simulink model "WindFarmDFIG"  (R2024a)
settings: Solver=FixedStepDiscrete  StartTime=0.0  StopTime=0.2  RelTol=1e-3
PreLoadFcn:
  | Ts=5e-6;
InitFcn:
  | xInitial = WindFarmDFIGInit;
  | Ts=5e-6;
undefined symbols (not defined in the file): D1, D11, Delta, DiscIntNeverNeededParam, find_system, level
libraries: powerlib_extras x38, spsThreePhaseVIMeasurementLib x6, simulink_extras x6, spsThreePhaseTransformerTwoWindingsLib x3, spsSeriesRLCBranchLib x2, spsUniversalBridgeLib x2, spsGroundLib x2, spsThreePhaseProgrammableVoltageSourceLib x1, spsThreePhaseMutualInductanceZ1Z0Lib x1, spsThreePhasePISectionLineLib x1, spsAsynchronousMachinepuUnitsLib x1, spsThreePhaseSeriesRLCBranchLib x1
(part 1 of 3)
settings Model: FPTRunName=Active  Creator=The MathWorks, Inc.  LastModifiedBy=TUF
settings SolverCC: AlgebraicLoopSolver=TrustRegion
settings DataIOCC: LimitDataPoints=on  LoadInitialState=on  SaveFormat=StructureWithTime  SaveOutput=off  SaveTime=off  ReturnWorkspaceOutputs=off
settings OptimizationCC: ExpressionDepthLimit=2147483647  InitFltsAndDblsToZero=on  LifeSpan=inf
settings DebuggingCC: SaveWithParameterizedLinksMsg=none  UnderspecifiedInitializationDetection=Classic  MergeDetectMultiDrivingBlocksExec=none  SignalResolutionControl=TryResolveAllWithWarning  SolverPrmCheckMsg=warning  FcnCallInpInsideContextMsg=warning  UnconnectedInputMsg=warning  UnconnectedOutputMsg=warning  StateNameClashWarn=warning  SubsystemReferenceDiagnosticForUnitTest=warning  SFUnexpectedBacktrackingDiag=warning  SFNoUnconditionalDefaultTransitionDiag=warning  SFExecutionAtInitializationDiag=none  ArithmeticOperatorsInVariantConditions=warning
settings HardwareCC: ProdBitPerPointer=32  ProdBitPerSizeT=32  ProdBitPerPtrDiffT=32  ProdLargestAtomicFloat=None  ProdIntDivRoundTo=Undefined  ProdEndianess=Unspecified  ProdWordSize=32  ProdHWDeviceType=32-bit Generic
settings ModelReferenceCC: EnableRefExpFcnMdlSchedulingChecks=on  PropagateSignalLabelsOutOfModel=off
settings SFSimCC: SimUseLocalCustomCode=off  CustomCodeUndefinedFunction=UseInterfaceOnly
settings RTWCC: RTWUseLocalCustomCode=off  GPUComputeCapability=3.5  DLArmComputeVersion=19.05
settings CodeAppCC: StateflowObjectComments=on
settings GRTTargetCC: TargetFcnLib=ansi_tfl_tmw.mat  TargetLangStandard=C89/C90 (ANSI)  CombineOutputUpdateFcns=off  GRTInterface=on
settings ConfigComp: CovMetricSettings=dw  CovSaveCumulativeToWorkspaceVar=on  CovSaveSingleToWorkspaceVar=on  CovExternalEMLEnable=off  CovSFcnEnable=off  CovBoundaryAbsTol=1.0e-5
settings SimscapeCC: SimscapeNormalizeSystem=off

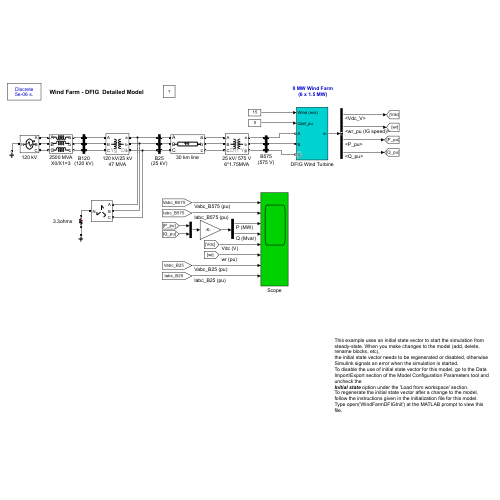
[thumbnail: Simulink's stored preview of the top-level diagram]
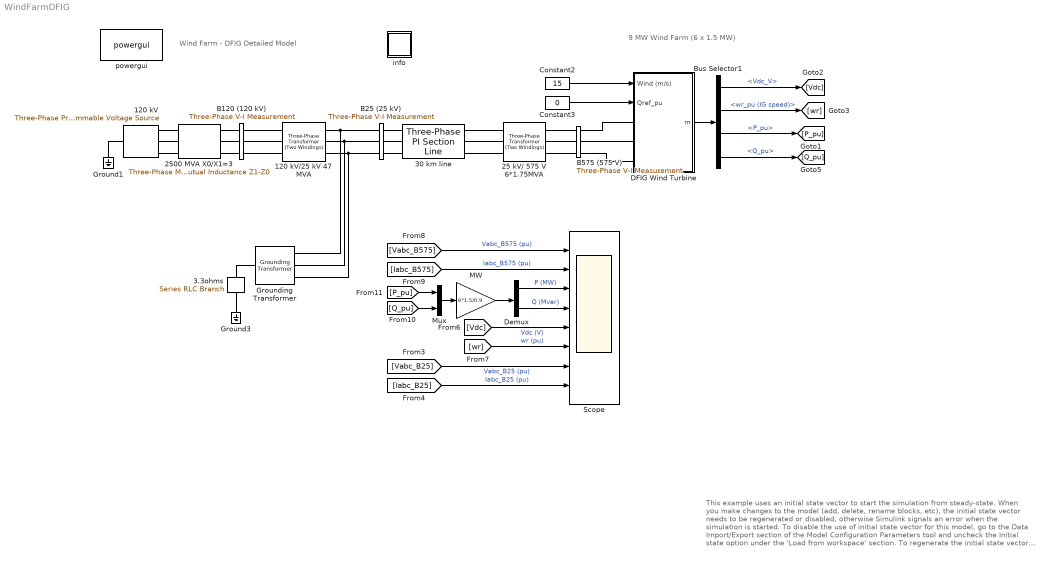
== system WindFarmDFIG ==
  note: 9 MW Wind Farm
      | (6 x 1.5 MW)
  note: Wind Farm - DFIG Detailed Model
  note: This example uses an initial state vector to start the simulation from steady-state. When you make changes to the model (add, delete, rename blocks, etc),
      | the initial state vector needs to be regenerated or disabled, otherwise Simulink signals an error when the simulation is started.
      | To disable the use of initial state vector for this model, go to the Data Import/Export section of the Model Configuration Parameters tool and uncheck the
      | Initial state option under the 'Load from workspace' section.
      | To regenerate the initial state vector after a change to the model, follow the instructions given in the initialization file for this model.
      | Type open('WindFarmDFIGInit') at the MATLAB prompt to view this file.
  120 kV : spsThreePhaseProgrammableVoltageSourceLib/Three-Phase Programmable Voltage Source  PositiveSequence=[120e3 0 60]  VariationEntity=Amplitude  VariationType=Table of time-amplitude pairs  VariationTypeAlt=Step  VariationStep=-0.2  VariationRate=10  VariationMagnitude=0.3  VariationFrequency=2  VariationTiming=[0.05 0.05+5/60]  VariationPhaseA=off  Amplitudes=[1 0.5 1.0]  TimeValues=[0 0.03 0.13]  HarmonicGeneration=off  HarmonicA=[1 -0.1 0 2]  HarmonicB=[2 0.15 35 2]*0  Timing="[0.1  2]"  BusType=swing  Pref=0  Qref=0  Qmin=-inf  Qmax=inf
  120 kV/25 kV 47 MVA : spsThreePhaseTransformerTwoWindingsLib/Three-Phase Transformer (Two Windings)  Winding1Connection=Yg  Winding2Connection=Delta (D1)  CoreType=Three single-phase transformers  SetSaturation=off  Hysteresis=off  DataFile='basic_model'  SetInitialFlux=off  Measurements=None  UNITS=pu  NominalPower=[47e6 60 ]  Winding1="[ 120e3  0.08/30   0.08 ]"  Winding2="[ 25e3  0.08/30  0.08]"  Rm=500  Lm=500  L0=0.5  Saturation="[ 0,0  ;  0.005,1.2  ;  1.0,1.4 ]"  InitialFluxes=[ 0.8 , -0.8 , 0.7 ]  BreakLoop=off  DiscreteSolver=Trapezoidal iterative  DataType=off  TransfoNumber=0
  25 kV/ 575 V 6*1.75MVA : spsThreePhaseTransformerTwoWindingsLib/Three-Phase Transformer (Two Windings)  Winding1Connection=Delta (D11)  Winding2Connection=Yg  CoreType=Three single-phase transformers  SetSaturation=off  Hysteresis=off  DataFile='hysteresis'  SetInitialFlux=off  Measurements=None  UNITS=pu  NominalPower="[1.75e6*6  60]"  Winding1=[25e3 , 0.025/30 , 0.025]  Winding2=[ 575, 0.025/30 , 0.025]  Rm=500  Lm=inf  L0=0.5  Saturation=[ 0,0 ; 0.0024,1.2 ; 1.0,1.52 ]  InitialFluxes=[ 0.8 , -0.8 , 0.7 ]  BreakLoop=off  DiscreteSolver=Trapezoidal iterative  DataType=off  TransfoNumber=0
  2500 MVA X0/X1=3 : spsThreePhaseMutualInductanceZ1Z0Lib/Three-Phase Mutual Inductance Z1-Z0  LConnTagsString=a|b|c  RConnTagsString=A|B|C  PositiveSequence="[0.1  1.0/(2*pi*60)] *120e3^2/2500e6"  ZeroSequence="[0.3  3.0/(2*pi*60)] *120e3^2/2500e6"
      settings: AttributesFormatString=\n
  "3.3ohms " : spsSeriesRLCBranchLib/Series RLC Branch  LConnTagsString=__new0  RConnTagsString=__new0  BranchType=R  Resistance=3.3  Inductance=[]  SetiL0=off  InitialCurrent=0  Capacitance=[]  Setx0=off  InitialVoltage=0  Measurements=None
  30 km line : spsThreePhasePISectionLineLib/Three-Phase PI Section Line  LConnTagsString=a|b|c  RConnTagsString=A|B|C  Length=30  Frequency=60  Resistances=[0.1153 0.413]  Inductances=[1.05e-3 3.32e-3]  Capacitances=[11.33e-009 5.01e-009]
  B120 (120 kV) : spsThreePhaseVIMeasurementLib/Three-Phase V-I Measurement  VoltageMeasurement=no  SetLabelV=off  LabelV=Vabc_B120  Vpu=off  VpuLL=off  CurrentMeasurement=no  SetLabelI=on  LabelI=Iabc_B120  Ipu=off  Pbase=100e6  Vbase=120e3  OutputType=Complex  PhasorSimulation=off  PSBequivalent=0
  B25 (25 kV) : spsThreePhaseVIMeasurementLib/Three-Phase V-I Measurement  VoltageMeasurement=phase-to-ground  SetLabelV=on  LabelV=Vabc_B25  Vpu=on  VpuLL=off  CurrentMeasurement=yes  SetLabelI=on  LabelI=Iabc_B25  Ipu=on  Pbase=10e6  Vbase=25e3  OutputType=Complex  PhasorSimulation=off  PSBequivalent=0
  B575 (575 V) : spsThreePhaseVIMeasurementLib/Three-Phase V-I Measurement  VoltageMeasurement=phase-to-ground  SetLabelV=on  LabelV=Vabc_B575  Vpu=on  VpuLL=off  CurrentMeasurement=yes  SetLabelI=on  LabelI=Iabc_B575  Ipu=on  Pbase=6*1.5e6/0.9  Vbase=575  OutputType=Complex  PhasorSimulation=off  PSBequivalent=0
  Bus Selector1 : BusSelector  OutputSignals=Vdc_V,wr_pu (IG speed),PQ_pu.P_pu,PQ_pu.Q_pu
  Constant2 : Constant  Value=15
  Constant3 : Constant  Value=0
  DFIG Wind Turbine : Subsystem  LoadFcn=%find_system(gcs,'FollowLinks', 'on', 'LookUnderMasks', 'all');  mask(DFIG Wind Turbine){Nb_wt=6, ShowParameters=Generator data for 1 wind turbine, nom=[1.5e6/.9 575 1975 60], sta=[ 0.023 0.18], rot=[ 0.016 0.16], Lm=2.9, mec=[0.685 0.01 3], init=[ -0.2,0   0,0,0   0,0,0 ], Imax_grid_conv=0.8, RL_grid=[ 0.3 0.003], Vdc_nom=1150, C_DClink1=10000e-6, C_var_filter1=120e3, Pmec1=1.5e6, wind_speed_CpMax=11, wind0=11, DisplayTurbChar=off, H_WT=4.32, Ksh=1.11, D_mutual=1.5, w_wt0=1.2, torque0=0.83, Kdc=[8   400], Kgrid_side_cur_reg=[0.83 5], Kspeed=[3 0.6], Krotor_side_cur_reg=[0.6 8], Ki_QV=[0.05 20], Kp_pitch=[150], Kcompensation=[3 30], PWM_freq_grid=2700, PWM_freq_rotor=1620, pitch_max=27, pitch_rate=10}
      mask prompts: Nb_wt "Number of wind turbines:"; ShowParameters "Display:"; nom "Nom. power, L-L volt. and freq. [Pn (VA), Vs_nom (Vrms), Vr_nom (Vrms), fn (Hz)]:"; sta "Stator [ Rs,Lls ] (p.u.):"; rot "Rotor [ Rr',Llr' ] (p.u.):"; Lm "Magnetizing inductance Lm (p.u.):"; mec "Inertia constant, friction factor, and pairs of poles [ H(s)  F(p.u.)  p ]:"; init "Initial conditions [s  th  ias  ibs  ics  phaseas phasebs phasecs]:"; Imax_grid_conv "Grid-side converter maximum current (pu of generator nominal current):"; RL_grid "Grid-side coupling inductor [ L, R] (p.u.):"; Vdc_nom "Nominal DC bus voltage (V):"; C_DClink1 "DC bus capacitor (F):"; C_var_filter1 "Line filter capacitor (Q=50) (var):"; Pmec1 "Nominal mechanical output power (W):"; wind_speed_CpMax "Wind speed at nominal speed and at Cp max (must be between 6 m/s and 30 m/s) (m/s):"; wind0 "Initial wind speed (m/s):"; DisplayTurbChar "Display wind turbine power characteristics:"; H_WT "Wind turbine inertia constant H (s):"; Ksh "Shaft spring constant refer to high-speed shaft (pu of nominal mechanical torque/rad):"; D_mutual "Shaft mutual damping (pu of nominal mechanical torque/pu dw):"; w_wt0 "Turbine initial speed (pu of nominal speed):"; torque0 "Initial output torque (pu of nominal mechanical torque):"; Kdc "DC bus voltage regulator gains [Kp Ki]:"; Kgrid_side_cur_reg "Grid-side converter current regulator gains [Kp Ki]:"; Kspeed "Speed regulator gains [Kp Ki]:"; Krotor_side_cur_reg "Rotor-side converter current regulator gains [Kp Ki]:"; Ki_QV "Q and V regulator gains [Ki_var Ki_volt]:"; Kp_pitch "Pitch controller gain [Kp]:"; Kcompensation "Pitch compensation gains [Kp Ki]:"; PWM_freq_grid "Frequency of the grid-side PWM carrier (Hz):"; PWM_freq_rotor "Frequency of the rotor-side PWM carrier (Hz):"; pitch_max "Maximum pitch angle (deg):"; pitch_rate "Maximum rate of change of pitch angle (deg/s):"
      mask help: This block implements a model of a variable speed pitch controlled wind turbine using a doubly-fed induction generator (DFIG).
      mask init:
      | %Generator data
      | Pnom=nom(1)*Nb_wt;
      | Vnom=nom(2);
      | Vnom_r=nom(3);
      | Fnom=nom(4);
      | Rs=sta(1);
      | Lls=sta(2);
      | Rr=rot(1);
      | Llr=rot(2);
      | H=mec(1);
      | F=mec(2);
      | p=mec(3);
      | 
      | % Converters data
      | L_RL=RL_grid(1);
      | R_RL=RL_grid(2);
      | Q_filter=50;
      | C_DClink=C_DClink1*Nb_wt;
      | C_var_filter=C_var_filter1*Nb_wt;
      | 
      | % Controller data
      | Freq_filter=1000*10;   %Hz
      | Zeta_filter=0.707;
      | Mod_index_max_grid=1.1;   %Maximum value of modulation index for grid-side converter
      | Mod_index_max_rotor=2;   %Maximum value of modulation index for rotor-side converter
      | Lim_grid_side_cur_reg=1.1; %Limit for grid-side PI current regulator (pu)
      | Lim_rotor_side_cur_reg=0.1; %Limit for rotor-side PI current regulator (pu)
      | Min_var_reg=0.9; %Minimum output value for integral var regulator (pu)
      | Max_var_reg=1.1; %Maximum output value for integral var regulator (pu)
      | Max_speed_reg=1; %Maximum output value for PI speed regulator (pu)
      | Kp_dc=Kdc(1);
      | Ki_dc=Kdc(2);
      | Kp_grid_side_cur_reg=Kgrid_side_cur_reg(1);
      | Ki_grid_side_cur_reg=Kgrid_side_cur_reg(2);
      | Kp_speed=Kspeed(1);
      | Ki_speed=Kspeed(2);
      | Kp_compensation=Kcompensation(1);
      | Ki_compensation=Kcompensation(2);
      | Kp_rotor_side_cur_reg=Krotor_side_cur_reg(1);
      | Ki_rotor_side_cur_reg=Krotor_side_cur_reg(2);
      | Ki_var=Ki_QV(1);
      | Ki_volt=Ki_QV(2);
      | Iq_ref_limit_time_constant=0.3; %(s)
      | T_speed=5;      %s
      | Min_mag_flux=0.5;   %(pu)
      | Max_Idr_ref=0.9;    %(pu)
      | Speed_max=1.2;  %(pu)
      | Speed_min=0.7;  %(pu)
      | Pitch_time_constant=0.01;    %(s)
      | 
      | 
      | % Turbine data
      | Pmec=Pmec1*Nb_wt;
      | c1 = 0.6450;
      | c2 = 116;
      | c3 = .4;
      | c4 = 5;
      | c5 = 21;
      | c6 = .00912;  % Set Pmin in stall condition (does not vary with wind_speed_Pmax)
      | c7 = .08;
      | c8 = .035;
      | theta=0;
      | CpMax=.5;
      | lambda_CpMax=9.9495;
      | 
      | c1_c8=[c1 c2 c3 c4 c5 c6 c7 c8];
      |   
      | 
      | %   Cp = c1*(c6*lambda + (-c4 - c3*(2.5 + theta) + c2*(1/(lambda + ...
      | %   c7*(2.5 + theta)) - c8/(1 + (2.5 + theta)^3)))/exp(c5*(1/(lambda + ...
      | %   c7*(2.5 + theta)) - c8/(1 + (2.5 + theta)^3))))
      | 
      | 
      |         %%%%%%%%%%%%%%%%%%%%%%%%%%%%%%%%%%%%%%%%%%%%%%%%%%%%%%%%%%%%%%%%%%%%%%%%%%%
      |         % Operation at Cp max
      |         %%%%%%%%%%%%%%%%%%%%%%%%%%%%%%%%%%%%%%%%%%%%%%%%%%%%%%%%%%%%%%%%%%%%%%%%%%%
      |         
      |         rated_omegar=1.2;
      |         omegar = rated_omegar;
      |         
      |         % Enforce boundaries on wind speed
      |         % A warning could be displayed
      |         if wind_speed_CpMax < 6
      |             wind_speed_CpMax=6;
      |             disp('Warning: Wind speed at nominal speed and at Cp max has been set to 6 m/s')
      |         end
      |         if wind_speed_CpMax > 30
      |             wind_speed_CpMax=30;
      |             disp('Warning: Wind speed at nominal speed and at Cp max has been set to 30 m/s')
      |         end
      | 
      |         K1=lambda_CpMax/omegar*wind_speed_CpMax;
      |         
      |         % Calculation of K2 needed to get P equal to the requested value at
      |         % Cp max for the requested wind speed
      |         
      |         Prated=Pmec1*Nb_wt;
      |         P_rated_omegar_theta_zero=0.75;
      |         
      |         K2 = P_rated_omegar_theta_zero*Prated/(wind_speed_CpMax^3*CpMax);
      |         
      |         K1_K2=[K1 K2];
      |         
      |         %%%%%%%%%%%%%%%%%%%%%%%%%%%%%%%%%%%%%%%%%%%%%%%%%%%%%%%%%%%%%%%%%%%%%%%%%%%
      |         % End of calculation for operation at Cp max
      |         %%%%%%%%%%%%%%%%%%%%%%%%%%%%%%%%%%%%%%%%%%%%%%%%%%%%%%%%%%%%%%%%%%%%%%%%%%%
      |         
      | 
      | %%%%%%%%%%%%%%%%%%%%%%%%%%%%%%%%%%%%%%%%%%%%%%%%%%%%%%%%%%%%%%%%%%%%%%%%%%%
      | % Plot turbine characteristics
      | %%%%%%%%%%%%%%%%%%%%%%%%%%%%%%%%%%%%%%%%%%%%%%%%%%%%%%%%%%%%%%%%%%%%%%%%%%% 
      | 
      | DisplayTurbChar=get_param(gcb,'DisplayTurbChar');
      | if strcmp(DisplayTurbChar,'on')
      |     vect_theta = 0:2:30;
      |     
      |     vect_lambda = 1:0.2:30;
      |     
      |     clear Cp;
      |     
      |     for i=1:length(vect_theta)
      |      for j=1:length(vect_lambda)
      |                 Cp(i,j) = c1*(c6*vect_lambda(j) + (-c4 - c3*(2.5 + vect_theta(i)) + c2*(1/(vect_lambda(j) + ...
      |                 c7*(2.5 + vect_theta(i))) - c8/(1 + (2.5 + vect_theta(i))^3)))/exp(c5*(1/(vect_lambda(j) + ...
      |                 c7*(2.5 + vect_theta(i))) - c8/(1 + (2.5 + vect_theta(i))^3))));
      |      end
      |     end
      | 
      |     figure(1);
      |     clf;
      |     hold on;
      | 
      |     plot(vect_lambda, Cp);
      |     axis([0, 25, 0, .6]);
      |     title('Wind Turbine Cp Characteristic (pitch angle increases by step of 2 deg.)');
      |     ylabel('Cp');
      |     set(gca,'ytick',[0 .1 .2 .3 .4 .5 .6]);
      |     xlabel('Lambda');
      |     grid on;
      |     text(10.1,0.51,'Pitch angle 0 degree');
      | 
      |     hold off
      |     
      |     % Plot of the wind turbine mechanical power output (pu) lambda and Cp
      |     % characteristics against wind speed (m/s) for a range of theta.
      |     
      |     wind_speed_range = [1,.2,30];
      |     vect_wind_speed = 1:0.2:30;
      |     
      |     clear lambda;
      |     clear Cp;
      |     clear P;
      | 
      |     for i=1:length(vect_theta)
      |         for j=1:length(vect_wind_speed)
      |             lambda(i,j) = K1*omegar/vect_wind_speed(j);
      |             Cp(i,j) = c1*(c6*lambda(i,j) + (-c4 - c3*(2.5 + vect_theta(i)) + c2*(1/(lambda(i,j) + ...
      |             c7*(2.5 + vect_theta(i))) - c8/(1 + (2.5 + vect_theta(i))^3)))/exp(c5*(1/(lambda(i,j) + ...
      |             c7*(2.5 + vect_theta(i))) - c8/(1 + (2.5 + vect_theta(i))^3))));
      |             P(i,j) = K2/Prated*vect_wind_speed(j)^3*Cp(i,j);
      |         end
      |     end
      |     
      |     
      |     figure(2);
      |     clf;
      |     hold on
      |     
      |     subplot(3,1,1);
      |     plot(vect_wind_speed, P);
      |     axis([0, 35, 0, 1.5]);
      |     title('Wind Turbine Characteristics (w = 1.2 pu, pitch angle increases by step of 2 deg.)');
      |     ylabel('P (pu)');
      |     set(gca,'ytick',0:.5:4);
      |     grid on;
      |     
      |     subplot(3,1,2);
      |     plot(vect_wind_speed, lambda);
      |     axis([0, 35, 0, 20]);
      |     ylabel('Lambda');
      |     grid on;
      |     
      |     subplot(3,1,3)
      |     plot(vect_wind_speed, Cp);
      |     axis([0, 35, 0, .6]);
      |     xlabel('Wind Speed (m/s)');
      |     ylabel('Cp');
      |     set(gca,'ytick',[0 .1 .2 .3 .4 .5 .6]);
      |     grid on;
      | 
      |     hold off
      |     set_param(gcb,'DisplayTurbChar','off')
      |     
      | end
      mask TypeOptions ShowParameters: Generator data for 1 wind turbine | Converters data for 1 wind turbine | Turbine data for 1 wind turbine | Drive train data for 1 wind turbine | Control parameters for 1 wind turbine
      mask Callback ShowParameters:
      | BlockName=getfullname(gcb);
      | %
      | Param_Show=get_param(BlockName,'ShowParameters');
      | Param_DisplayTurbChar=get_param(BlockName,'DisplayTurbChar');
      | 
      | p_mask{3}='off';p_mask{4}='off';p_mask{5}='off';
      | p_mask{6}='off';p_mask{7}='off';p_mask{8}='off';p_mask{9}='off';
      | p_mask{10}='off';p_mask{11}='off';p_mask{12}='off';p_mask{13}='off';
      | p_mask{14}='off';p_mask{15}='off';p_mask{16}='off';p_mask{17}='off';
      | p_mask{18}='off';p_mask{19}='off';p_mask{20}='off';p_mask{21}='off';
      | p_mask{22}='off';p_mask{23}='off';p_mask{24}='off';p_mask{25}='off';
      | p_mask{26}='off';p_mask{27}='off';p_mask{28}='off';p_mask{29}='off';
      | p_mask{30}='off';p_mask{31}='off';p_mask{32}='off';p_mask{33}='off';
      | 
      | 
      | switch Param_Show
      | 	case 'Generator data for 1 wind turbine'
      | 		p_mask{3}='on';p_mask{4}='on';p_mask{5}='on'; p_mask{6}='on';
      |         p_mask{7}='on'; p_mask{8}='on';
      |     case 'Converters data for 1 wind turbine'
      | 		p_mask{9}='on';p_mask{10}='on';p_mask{11}='on';p_mask{12}='on';
      |         p_mask{13}='on';
      | 	case 'Turbine data for 1 wind turbine'
      |         p_mask{14}='on';p_mask{15}='on';p_mask{16}='on';p_mask{17}='on';
      |     case 'Drive train data for 1 wind turbine'
      |         p_mask{18}='on';p_mask{19}='on';p_mask{20}='on';p_mask{21}='on';
      |         p_mask{22}='on';
      |     case 'Control parameters for 1 wind turbine'
      |         p_mask{23}='on';p_mask{24}='on';p_mask{25}='on';
      |         p_mask{26}='on';p_mask{27}='on';p_mask{28}='on';p_mask{29}='on';
      |         p_mask{30}='on'; p_mask{31}='on';p_mask{32}='on'; p_mask{33}='on';
      | end
      | 
      | ParVisible={'on','on',p_mask{3},p_mask{4},p_mask{5},p_mask{6},p_mask{7},...
      |     p_mask{8},p_mask{9},p_mask{10},p_mask{11},p_mask{12},p_mask{13},...
      |     p_mask{14},p_mask{15},p_mask{16},p_mask{17},p_mask{18},p_mask{19},...
      |     p_mask{20},p_mask{21},p_mask{22},p_mask{23},p_mask{24},p_mask{25},...
      |     p_mask{26},p_mask{27},p_mask{28},p_mask{29},p_mask{30},p_mask{31},...
      |     p_mask{32},p_mask{33}};
      | %
      | set_param(BlockName,'MaskVisibilities',ParVisible);
      | set_param(BlockName,'DisplayTurbChar',Param_DisplayTurbChar);
  Demux : Demux  Outputs=2
  Ground1 : spsGroundLib/Ground  LConnTagsString=a
  Ground3 : spsGroundLib/Ground  LConnTagsString=a
  "Grounding Transformer " : spsGroundingTransformerLib/Grounding Transformer   UNITS=pu  NominalPower="[100e6   60]"  NominalVoltage=25e3  ZeroSequenceImpedance_pu=[0.025 0.75]  MagnetizationBranch_pu=[500 500]  ZeroSequenceImpedance_SI=[0.052083 589.05]  MagnetizationBranch_SI=[1041.7 3.927e+005]  Measurements=None
  MW : Gain  Gain=6*1.5/0.9  SaturateOnIntegerOverflow=on  OutDataTypeStr=Inherit: Same as input  ParamDataTypeStr=Inherit: Same as input
  Mux : Mux  Inputs=2
  Scope : Scope  NumInputPorts=8
  info : Subsystem
      settings: OpenFcn="showExample(\"simscapeelectricalsps/WindFarmDFIGExample\")"
      mask Display: disp('?')
  powergui : spspowerguiLib/powergui  SimulationMode=Discrete  SampleTime=Ts  frequency=60  Iterations=50  frequencyindice=60  Pbase=100e6  ErrMax=1e-4  UnitsV=kV  UnitsW=MW  buscounter=0  FunctionMessages=off  echomessages=off  EnableUseOfTLC=off  CurrentSourceSwitches=off  DisableSnubberDevices=off  DisableRonSwitches=off  DisableVfSwitches=off  DisplayEquations=off  AutomaticDiscreteSolvers=off  SolverType=Tustin/Backward Euler (TBE)  Interpol=off  ExternalGateDelay=off  methode=off  Ts=0  x0status=blocks  SPID=off  SwTol=0  HookPort=off  NonlinearTolerance=1e-4  nMaxIteration=100  ContinueOnMaxIteration=off  RestoreLinks=warning  ResistiveCurrentMeasurement=off  Frange=[0:0.1:90]  Ylog=off  Xlog=off  ShowGrid=off  save=on  variable=ZData  structure=Vabc_Iabc  ZoomFFT=on  StartTime=0.0  cycles=1  DisplayStyle=1  fundamental=60  FreqAxis=off  MaxFrequency=1000  frequencyindicesteady=1  RmsSteady=1  display=off
  wires:
  [Vabc_B575] -> Scope/1  "Vabc_B575 (pu)"
  [Iabc_B575] -> Scope/2  "Iabc_B575 (pu)"
  Demux/1 -> Scope/3  "P (MW)"
  Demux/2 -> Scope/4  "Q (Mvar)"
  [Vdc] -> Scope/5  "Vdc (V)"
  [wr] -> Scope/6  "wr (pu)"
  [Vabc_B25] -> Scope/7  "Vabc_B25 (pu)"
  [Iabc_B25] -> Scope/8  "Iabc_B25 (pu)"
  [Q_pu] -> Mux/2
  [P_pu] -> Mux/1
  Mux/1 -> MW/1
  MW/1 -> Demux/1
  Constant2/1 -> DFIG Wind Turbine/1("Wind (m/s) ")
  Constant3/1 -> DFIG Wind Turbine/2(Qref_pu)
  DFIG Wind Turbine/1(m) -> Bus Selector1/1
  Bus Selector1/1 -> [Vdc]  "<Vdc_V>"
  Bus Selector1/2 -> [wr]  "<wr_pu (IG speed)>"
  Bus Selector1/3 -> [P_pu]  "<P_pu>"
  Bus Selector1/4 -> [Q_pu]  "<Q_pu>"
  connections:
  120 kV/25 kV 47 MVA/RConn3 -- B25 (25 kV)/LConn3 -- "Grounding Transformer "/LConn3
  Ground1/LConn1 -- 120 kV/LConn1
  120 kV/RConn1 -- 2500 MVA X0/X1=3/LConn1
  120 kV/RConn2 -- 2500 MVA X0/X1=3/LConn2
  120 kV/RConn3 -- 2500 MVA X0/X1=3/LConn3
  B120 (120 kV)/LConn1 -- 2500 MVA X0/X1=3/RConn1
  B120 (120 kV)/LConn2 -- 2500 MVA X0/X1=3/RConn2
  B120 (120 kV)/LConn3 -- 2500 MVA X0/X1=3/RConn3
  120 kV/25 kV 47 MVA/LConn1 -- B120 (120 kV)/RConn1
  120 kV/25 kV 47 MVA/LConn2 -- B120 (120 kV)/RConn2
  120 kV/25 kV 47 MVA/LConn3 -- B120 (120 kV)/RConn3
  B25 (25 kV)/RConn1 -- 30 km line/LConn1
  B25 (25 kV)/RConn2 -- 30 km line/LConn2
  B25 (25 kV)/RConn3 -- 30 km line/LConn3
  120 kV/25 kV 47 MVA/RConn1 -- B25 (25 kV)/LConn1 -- "Grounding Transformer "/LConn1
  120 kV/25 kV 47 MVA/RConn2 -- B25 (25 kV)/LConn2 -- "Grounding Transformer "/LConn2
  "3.3ohms "/RConn1 -- Ground3/LConn1
  30 km line/RConn1 -- 25 kV/ 575 V 6*1.75MVA/LConn1
  30 km line/RConn2 -- 25 kV/ 575 V 6*1.75MVA/LConn2
  30 km line/RConn3 -- 25 kV/ 575 V 6*1.75MVA/LConn3
  "3.3ohms "/LConn1 -- "Grounding Transformer "/RConn1
  25 kV/ 575 V 6*1.75MVA/RConn1 -- B575 (575 V)/LConn1
  25 kV/ 575 V 6*1.75MVA/RConn2 -- B575 (575 V)/LConn2
  25 kV/ 575 V 6*1.75MVA/RConn3 -- B575 (575 V)/LConn3
  DFIG Wind Turbine/LConn2 -- B575 (575 V)/RConn2
  DFIG Wind Turbine/LConn1 -- B575 (575 V)/RConn1
  DFIG Wind Turbine/LConn3 -- B575 (575 V)/RConn3

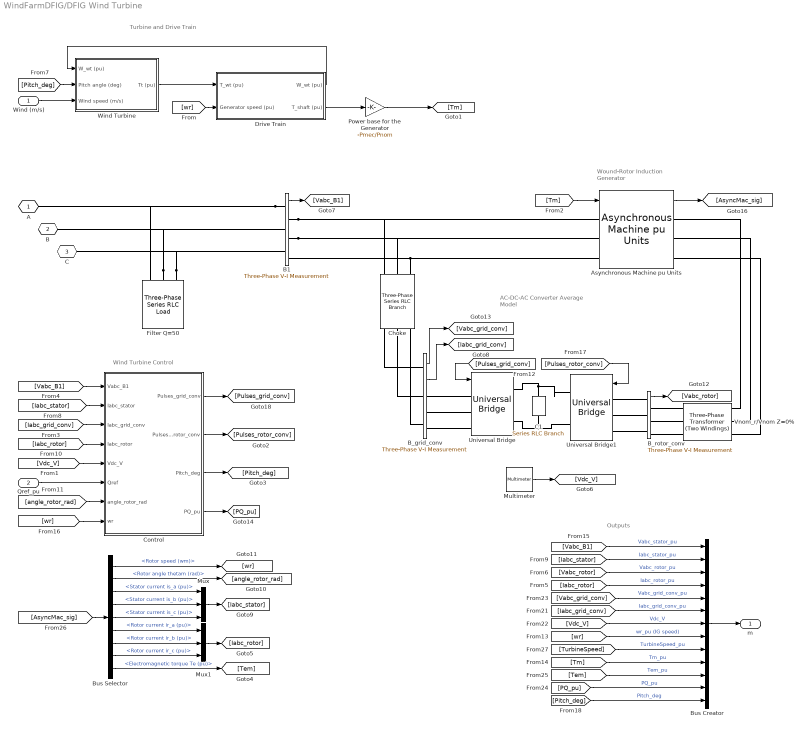
== system WindFarmDFIG/DFIG Wind Turbine ==
  note: Turbine and Drive Train
  note: Wind Turbine Control
  note: Wound-Rotor
      | Induction Generator
  note: AC-DC-AC Converter
      | Average Model
  note: Outputs
  "Wind (m/s) " : Inport
  Qref_pu : Inport  Port=2
  Asynchronous Machine pu Units : spsAsynchronousMachinepuUnitsLib/Asynchronous Machine pu Units  RotorType=Wound  PresetModel=No  MechanicalLoad=Torque Tm  ShowDetailedParameters=on  ReferenceFrame=Rotor  Units=pu  MeasurementBus=off  NominalParameters=[ Pnom Vnom Fnom ]  VoltageRatio=1  Stator=[ Rs Lls]  Rotor=[ Rr Llr]  Cage1=[0.01909 0.0397]  Cage2=[0.01909 0.0397]  Lm=Lm  Mechanical=[H F p]  PolePairs=3  InitialConditions=init  SimulateSaturation=off  Saturation="[0.212,0.4201,0.8125,1.0979,1.4799,2.2457,3.2586,4.5763,6.4763 ;   0.5,0.7,0.9,1,1.1,1.2 ,1.3,1.4,1.5]"  LoadFlowParameters=0  TsPowergui=0  TsBlock=-1  IterativeModel=Trapezoidal non iterative  IterativeDiscreteModel=Trapezoidal non iterative  Pmec=0
  B1 : spsThreePhaseVIMeasurementLib/Three-Phase V-I Measurement  VoltageMeasurement=phase-to-ground  SetLabelV=off  LabelV=Vabc  Vpu=on  VpuLL=off  CurrentMeasurement=no  SetLabelI=on  LabelI=Iabc_B1  Ipu=on  Pbase=Pnom  Vbase=Vnom  OutputType=Complex  PhasorSimulation=off  PSBequivalent=0
  B_grid_conv : spsThreePhaseVIMeasurementLib/Three-Phase V-I Measurement  VoltageMeasurement=phase-to-ground  SetLabelV=off  LabelV=Vabc_B1  Vpu=on  VpuLL=off  CurrentMeasurement=yes  SetLabelI=off  LabelI=Iabc  Ipu=on  Pbase=Pnom  Vbase=Vnom  OutputType=Complex  PhasorSimulation=off  PSBequivalent=0
  B_rotor_conv : spsThreePhaseVIMeasurementLib/Three-Phase V-I Measurement  VoltageMeasurement=phase-to-phase  SetLabelV=off  LabelV=Vabc_B1  Vpu=on  VpuLL=off  CurrentMeasurement=no  SetLabelI=off  LabelI=Iabc  Ipu=on  Pbase=Pnom  Vbase=Vnom_r  OutputType=Complex  PhasorSimulation=off  PSBequivalent=0
  Bus Creator : BusCreator  Inputs=13
  Bus Selector : BusSelector  OutputSignals=Mechanical.Rotor speed (wm),Mechanical.Rotor angle thetam (rad),Stator measurements.Stator current is_a (pu),Stator measurements.Stator current is_b (pu),Stator measurements.Stator current is_c (pu),Rotor measurements.Rotor current ir_a (pu),Rotor measurements.Rotor current ir_b (pu),Rotor measurements.Rotor current ir_c (pu),Mechanical.Electromagnetic torque Te (pu)
  C1 : spsSeriesRLCBranchLib/Series RLC Branch  LConnTagsString=__new0  RConnTagsString=__new0  BranchType=C  Resistance=[]  Inductance=[]  SetiL0=off  InitialCurrent=0  Capacitance=C_DClink  Setx0=on  InitialVoltage=Vdc_nom  Measurements=Branch voltage
  "Choke " : spsThreePhaseSeriesRLCBranchLib/Three-Phase Series RLC Branch  LConnTagsString=A|B|C  RConnTagsString=A|B|C  BranchType=RL  Resistance=R_RL*Vnom^2/Pnom  Inductance=L_RL*Vnom^2/Pnom/(2*pi*Fnom)  Capacitance=[]  Measurements=None
  Control : Subsystem
  Drive Train : Subsystem  mask(Wind Turbine shaft){H_WT=H_WT, Ksh=Ksh, D_mutual=D_mutual, wbase=2*pi*Fnom/p, w_wt0=w_wt0, torque0=torque0, Ts=Ts}
      mask prompts: H_WT "Wind turbine inertia constant H (s):"; Ksh "Shaft spring constant (pu of nominal mechanical torque/rad):"; D_mutual "Shaft mutual damping (pu of nominal mechanical torque/pu dw):"; wbase "Shaft base speed (rad/s):"; w_wt0 "Turbine initial speed (pu of base speed):"; torque0 "Initial output torque (pu of nominal mechanical torque):"; Ts "Sample time (s):"
      mask help:
      | This block implements a wind turbine drive train model. All shaft parameters are referred to high-speed shaft (generator shaft).
      |
      | The first input is the wind turbine torque in per unit (pu) based on the nominal power of the turbine and the base speed of the generator. The second input is the generator speed in pu based on the base speed of the generator.
      |
      | The outputs are:
      | 1- the transmitted torque of the shaft in pu based on the nominal power of the turbine and the base speed of the generator.
      | 2- the wind turbine speed in pu of the base speed of the generator.
  Filter Q=50 : spsThreePhaseSeriesRLCLoadLib/Three-Phase Series RLC Load  LConnTagsString=A|B|C  Configuration=Y (grounded)  NominalVoltage=Vnom  Vabc=[1e3 1e3 1e3]  Vabcp=[1e3 1e3 1e3]  NominalFrequency=Fnom  UnbalancedPower=off  ActivePower=C_var_filter/Q_filter  InductivePower=0  CapacitivePower=C_var_filter  Pabc=[10e3 9e3 11e3]  QLabc=[100 90 110]  QCabc=[100 90 110]  Pabcp=[10e3 9e3 11e3]  QLabcp=[100 90 110]  QCabcp=[100 90 110]  Measurements=None  LoadType=constant Z
  Multimeter : spsMultimeterLib/Multimeter  L=1  sel=1  yselected={}  Gain=1  OutputType=Complex  PlotAtSimulationStop=off  PhasorSimulation=off
  Mux : Mux  Inputs=3
  Mux1 : Mux  Inputs=3
  Power base for the Generator : Gain  Gain=-Pmec/Pnom  SaturateOnIntegerOverflow=on  OutDataTypeStr=Inherit: Same as input  ParamDataTypeStr=Inherit: Same as input
  Universal Bridge : spsUniversalBridgeLib/Universal Bridge  Arms=3  SnubberResistance=1e3  SnubberCapacitance=inf  Device=IGBT / Diodes  Ron=1e-4/Nb_wt  Lon=0  ForwardVoltages="[  0  0  ]"  ForwardVoltage=0  GTOparameters=[ 10e-6 , 20e-6 ]  IGBTparameters=[ 0 , 0 ]  Measurements=None  Measurements_2=None  converterType=Rectifier
  Universal Bridge1 : spsUniversalBridgeLib/Universal Bridge  Arms=3  SnubberResistance=1e3  SnubberCapacitance=inf  Device=IGBT / Diodes  Ron=1e-4/Nb_wt  Lon=0  ForwardVoltages="[  0  0  ]"  ForwardVoltage=0  GTOparameters=[ 10e-6 , 20e-6 ]  IGBTparameters=[ 0 , 0 ]  Measurements=None  Measurements_2=None  converterType=Rectifier
  Vnom_r/Vnom Z=0% : spsThreePhaseTransformerTwoWindingsLib/Three-Phase Transformer (Two Windings)  Winding1Connection=Y  Winding2Connection=Y  CoreType=Three single-phase transformers  SetSaturation=off  Hysteresis=off  DataFile='hysteresis'  SetInitialFlux=off  Measurements=None  UNITS=pu  NominalPower=[ Pnom , Fnom ]  Winding1=[ Vnom_r , 0, 0]  Winding2=[ Vnom , 0, 0]  Rm=500  Lm=inf  L0=0.5  Saturation=[ 0,0 ; 0.0024,1.2 ; 1.0,1.52 ]  InitialFluxes=[ 0.8 , -0.8 , 0.7 ]  BreakLoop=off  DiscreteSolver=Trapezoidal iterative  DataType=off  TransfoNumber=0
  Wind Turbine : Subsystem  mask(Wind Turbine){Prated=Pmec, c1_c8=c1_c8, K1_K2=K1_K2, wind0=wind0, Ts=Ts}
      mask prompts: Prated "Nominal mechanical output power (W):"; c1_c8 "Coefficients [c1 ... c8]"; K1_K2 "Parameters [K1 K2]"; wind0 "Initial wind speed (m/s):"; Ts "Sample time (s):"
      mask help:
      | This block implements a generic wind turbine models.
      |
      | The first input is the turbine speed in per unit of the generator base speed. For a synchronous or asynchronous generator, the base speed is the synchronous speed. For a permanent-magnet generator, the base speed is defined as the speed producing nominal voltage at  no load. The second input is the blade pitch angle in degrees. The third input is the wind speed in m/s.
      |
      | The output is the torque applied to the drive train in per unit based on the nominal power of the turbine and the base speed of the generator.
      mask init:
      | c1 = c1_c8(1);
      | c2 = c1_c8(2);
      | c3 = c1_c8(3);
      | c4 = c1_c8(4);
      | c5 = c1_c8(5);
      | c6 = c1_c8(6);
      | c7 = c1_c8(7);;
      | c8 = c1_c8(8);
      | 
      | K1=K1_K2(1);
      | K2=K1_K2(2);
      settings: OpenFcn=power_openblockproxy();
      mask Display: disp('');
  A : PMIOPort  Tag=PMCPort  Side=Left
  B : PMIOPort  Tag=PMCPort  Port=2  Side=Left
  C : PMIOPort  Tag=PMCPort  Port=3  Side=Left
  m : Outport  VectorParamsAs1DForOutWhenUnconnected=off
  wires:
  [Pulses_rotor_conv] -> Universal Bridge1/1
  [Pulses_grid_conv] -> Universal Bridge/1
  Multimeter/1 -> [Vdc_V]
  [Pitch_deg] -> Bus Creator/13  "Pitch_deg"
  [PQ_pu] -> Bus Creator/12  "PQ_pu"
  Control/4(PQ_pu) -> [PQ_pu]
  [Tem] -> Bus Creator/11  "Tem_pu"
  [Tm] -> Bus Creator/10  "Tm_pu"
  [TurbineSpeed] -> Bus Creator/9  "TurbineSpeed_pu"
  [Vdc_V] -> Bus Creator/7  "Vdc_V"
  [Iabc_grid_conv] -> Bus Creator/6  "Iabc_grid_conv_pu"
  [Vabc_grid_conv] -> Bus Creator/5  "Vabc_grid_conv_pu"
  [Iabc_rotor] -> Bus Creator/4  "Iabc_rotor_pu"
  [Vabc_rotor] -> Bus Creator/3  "Vabc_rotor_pu"
  [Iabc_stator] -> Bus Creator/2  "Iabc_stator_pu"
  [Vabc_B1] -> Bus Creator/1  "Vabc_stator_pu"
  Asynchronous Machine pu Units/1 -> [AsyncMac_sig]
  Control/2(Pulses_rotor_conv) -> [Pulses_rotor_conv]
  [Pitch_deg] -> Wind Turbine/2(Pitch angle (deg))
  Drive Train/1(W_wt (pu)) -> Wind Turbine/1(W_wt (pu))
  "Wind (m/s) "/1 -> Wind Turbine/3(Wind speed (m/s))
  Power base for the Generator/1 -> [Tm]
  Drive Train/2(T_shaft (pu)) -> Power base for the Generator/1
  [wr] -> Drive Train/2(Generator speed (pu))
  Wind Turbine/1(Tt (pu)) -> Drive Train/1(T_wt (pu))
  Qref_pu/1 -> Control/6(Qref)
  Bus Selector/9 -> [Tem]  "<Electromagnetic torque Te (pu)>"
  Bus Selector/1 -> [wr]  "<Rotor speed (wm)>"
  Bus Creator/1 -> m/1
  B_rotor_conv/1 -> [Vabc_rotor]
  B1/1 -> [Vabc_B1]
  [Vabc_B1] -> Control/1(Vabc_B1)
  [Iabc_grid_conv] -> Control/3(Iabc_grid_conv)
  [Iabc_rotor] -> Control/4(Iabc_rotor)
  [angle_rotor_rad] -> Control/7(angle_rotor_rad)
  Mux1/1 -> [Iabc_rotor]
  Mux/1 -> [Iabc_stator]
  [Vdc_V] -> Control/5(Vdc_V)
  Control/3(Pitch_deg) -> [Pitch_deg]
  [Iabc_stator] -> Control/2(Iabc_stator)
  [wr] -> Control/8(wr)
  Bus Selector/8 -> Mux1/3  "<Rotor current ir_c (pu)>"
  Bus Selector/7 -> Mux1/2  "<Rotor current ir_b (pu)>"
  Bus Selector/6 -> Mux1/1  "<Rotor current ir_a (pu)>"
  Bus Selector/5 -> Mux/3  "<Stator current is_c (pu)>"
  Bus Selector/4 -> Mux/2  "<Stator current is_b (pu)>"
  Bus Selector/3 -> Mux/1  "<Stator current is_a (pu)>"
  Bus Selector/2 -> [angle_rotor_rad]  "<Rotor angle thetam (rad)>"
  B_grid_conv/2 -> [Iabc_grid_conv]
  B_grid_conv/1 -> [Vabc_grid_conv]
  Control/1(Pulses_grid_conv) -> [Pulses_grid_conv]
  [AsyncMac_sig] -> Bus Selector/1
  [wr] -> Bus Creator/8  "wr_pu (IG speed)"
  [Tm] -> Asynchronous Machine pu Units/1
  connections:
  Universal Bridge1/LConn3 -- B_rotor_conv/LConn3
  Universal Bridge1/LConn2 -- B_rotor_conv/LConn2
  Universal Bridge1/LConn1 -- B_rotor_conv/LConn1
  C1/LConn1 -- Universal Bridge/RConn1 -- Universal Bridge1/RConn1
  B_grid_conv/RConn2 -- Universal Bridge/LConn2
  B_grid_conv/RConn1 -- Universal Bridge/LConn1
  B_grid_conv/RConn3 -- Universal Bridge/LConn3
  C1/RConn1 -- Universal Bridge/RConn2 -- Universal Bridge1/RConn2
  Filter Q=50/LConn3 -- B1/LConn3 -- C/RConn1
  Filter Q=50/LConn2 -- B1/LConn2 -- B/RConn1
  B1/LConn1 -- Filter Q=50/LConn1 -- A/RConn1
  B_rotor_conv/RConn3 -- Vnom_r/Vnom Z=0%/LConn3
  B_rotor_conv/RConn2 -- Vnom_r/Vnom Z=0%/LConn2
  B_rotor_conv/RConn1 -- Vnom_r/Vnom Z=0%/LConn1
  B1/RConn3 -- "Choke "/LConn3 -- Asynchronous Machine pu Units/LConn3
  B1/RConn1 -- "Choke "/LConn1 -- Asynchronous Machine pu Units/LConn1
  Asynchronous Machine pu Units/RConn3 -- Vnom_r/Vnom Z=0%/RConn3
  Asynchronous Machine pu Units/RConn1 -- Vnom_r/Vnom Z=0%/RConn1
  Asynchronous Machine pu Units/RConn2 -- Vnom_r/Vnom Z=0%/RConn2
  "Choke "/RConn3 -- B_grid_conv/LConn3
  "Choke "/RConn2 -- B_grid_conv/LConn2
  "Choke "/RConn1 -- B_grid_conv/LConn1
  B1/RConn2 -- "Choke "/LConn2 -- Asynchronous Machine pu Units/LConn2

== system WindFarmDFIG/info ==

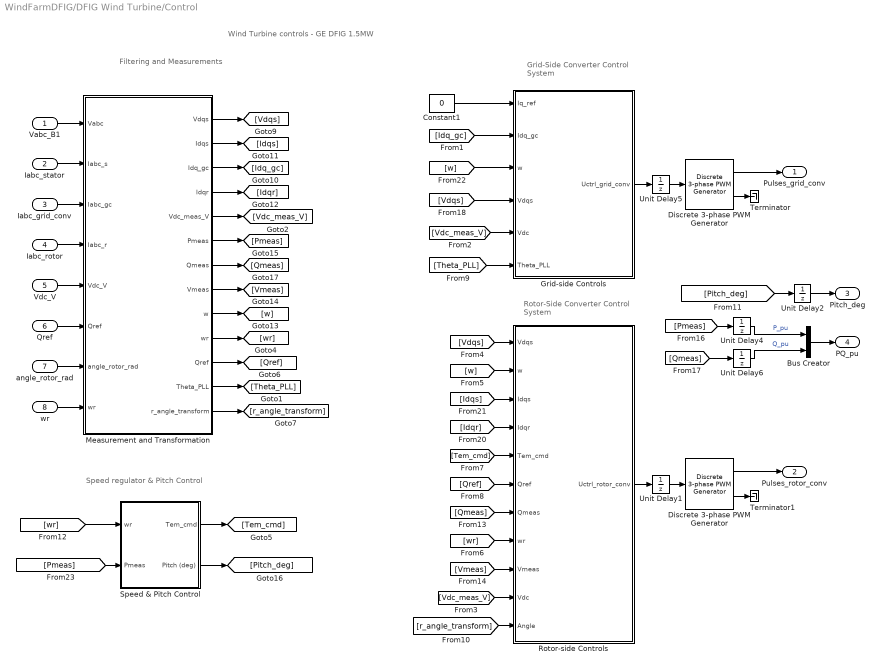
== system WindFarmDFIG/DFIG Wind Turbine/Control ==
  note: Speed regulator & Pitch Control
  note: Grid-Side Converter
      | Control System
  note: Rotor-Side Converter
      | Control System
  note: Filtering and
      | Measurements
  note: Wind Turbine controls - GE DFIG 1.5MW
  Vabc_B1 : Inport
  Iabc_stator : Inport  Port=2
  Iabc_grid_conv : Inport  Port=3
  Iabc_rotor : Inport  Port=4
  Vdc_V : Inport  Port=5
  Qref : Inport  Port=6
  angle_rotor_rad : Inport  Port=7
  wr : Inport  Port=8
  Bus Creator : BusCreator  Inputs=2
  Constant1 : Constant  Value=0
  Discrete 3-phase PWM Generator : powerlib_extras/Discrete  Control Blocks/Discrete 3-phase PWM Generator  ModulatorType=2-level  ModulatorMode=Un-synchronized  nF=27  Fc=PWM_freq_grid  ModulatingSignals=off  m=0.2  Freq=60  Phase=0  Ts=Ts
  "Discrete 3-phase PWM Generator " : powerlib_extras/Discrete  Control Blocks/Discrete 3-phase PWM Generator  ModulatorType=2-level  ModulatorMode=Un-synchronized  nF=27  Fc=PWM_freq_rotor  ModulatingSignals=off  m=0.2  Freq=60  Phase=0  Ts=Ts
  Grid-side Controls : Subsystem
  Measurement and Transformation : Subsystem
  Rotor-side Controls : Subsystem
  Speed & Pitch Control : Subsystem
  Terminator : Terminator
  Terminator1 : Terminator
  Unit Delay{1..2,4..6} (5 alike) : UnitDelay  SampleTime=Ts  HasFrameUpgradeWarning=on
  Pulses_grid_conv : Outport  VectorParamsAs1DForOutWhenUnconnected=off
  Pulses_rotor_conv : Outport  Port=2  VectorParamsAs1DForOutWhenUnconnected=off
  Pitch_deg : Outport  Port=3  VectorParamsAs1DForOutWhenUnconnected=off
  PQ_pu : Outport  Port=4  VectorParamsAs1DForOutWhenUnconnected=off
  wires:
  Unit Delay6/1 -> Bus Creator/2  "Q_pu"
  Unit Delay4/1 -> Bus Creator/1  "P_pu"
  Unit Delay2/1 -> Pitch_deg/1
  Unit Delay1/1 -> "Discrete 3-phase PWM Generator "/1
  Unit Delay5/1 -> Discrete 3-phase PWM Generator/1
  "Discrete 3-phase PWM Generator "/2 -> Terminator1/1
  Discrete 3-phase PWM Generator/2 -> Terminator/1
  "Discrete 3-phase PWM Generator "/1 -> Pulses_rotor_conv/1
  Discrete 3-phase PWM Generator/1 -> Pulses_grid_conv/1
  Rotor-side Controls/1(Uctrl_rotor_conv) -> Unit Delay1/1
  Grid-side Controls/1(Uctrl_grid_conv) -> Unit Delay5/1
  [Qmeas] -> Unit Delay6/1
  [Pmeas] -> Unit Delay4/1
  Bus Creator/1 -> PQ_pu/1
  Speed & Pitch Control/1(Tem_cmd) -> [Tem_cmd]
  Speed & Pitch Control/2(Pitch (deg)) -> [Pitch_deg]
  [r_angle_transform] -> Rotor-side Controls/11(Angle)
  [Vdc_meas_V] -> Rotor-side Controls/10(Vdc)
  Measurement and Transformation/13(r_angle_transform) -> [r_angle_transform]
  [Theta_PLL] -> Grid-side Controls/6(Theta_PLL)
  Measurement and Transformation/12(Theta_PLL) -> [Theta_PLL]
  [Vmeas] -> Rotor-side Controls/9(Vmeas)
  Measurement and Transformation/8(Vmeas) -> [Vmeas]
  [Qmeas] -> Rotor-side Controls/7(Qmeas)
  Measurement and Transformation/7(Qmeas) -> [Qmeas]
  Vabc_B1/1 -> Measurement and Transformation/1(Vabc)
  Iabc_grid_conv/1 -> Measurement and Transformation/3(Iabc_gc)
  Iabc_rotor/1 -> Measurement and Transformation/4(Iabc_r)
  Iabc_stator/1 -> Measurement and Transformation/2(Iabc_s)
  angle_rotor_rad/1 -> Measurement and Transformation/7(angle_rotor_rad)
  Constant1/1 -> Grid-side Controls/1(Iq_ref)
  Measurement and Transformation/1(Vdqs) -> [Vdqs]
  Measurement and Transformation/2(Idqs) -> [Idqs]
  Measurement and Transformation/3(Idq_gc) -> [Idq_gc]
  Measurement and Transformation/4(Idqr) -> [Idqr]
  Measurement and Transformation/6(Pmeas) -> [Pmeas]
  Measurement and Transformation/9(w) -> [w]
  [Idq_gc] -> Grid-side Controls/2(Idq_gc)
  [w] -> Grid-side Controls/3(w)
  [Vdqs] -> Grid-side Controls/4(Vdqs)
  [Vdc_meas_V] -> Grid-side Controls/5(Vdc)
  [Vdqs] -> Rotor-side Controls/1(Vdqs)
  [w] -> Rotor-side Controls/2(w)
  [Idqs] -> Rotor-side Controls/3(Idqs)
  [Idqr] -> Rotor-side Controls/4(Idqr)
  [Tem_cmd] -> Rotor-side Controls/5(Tem_cmd)
  [Qref] -> Rotor-side Controls/6(Qref)
  [wr] -> Speed & Pitch Control/1(wr)
  Measurement and Transformation/5(Vdc_meas_V) -> [Vdc_meas_V]
  Measurement and Transformation/10("wr ") -> [wr]
  Measurement and Transformation/11("Qref ") -> [Qref]
  Vdc_V/1 -> Measurement and Transformation/5(Vdc_V)
  Qref/1 -> Measurement and Transformation/6(Qref)
  wr/1 -> Measurement and Transformation/8(wr)
  [Pmeas] -> Speed & Pitch Control/2(Pmeas)
  [Pitch_deg] -> Unit Delay2/1
  [wr] -> Rotor-side Controls/8(wr)

== system WindFarmDFIG/DFIG Wind Turbine/Drive Train ==
  note: Shaft
  note: Turbine
  note: Wind turbine drive train based on a 2-masse model
  T_wt (pu) : Inport
  Generator speed (pu) : Inport  Port=2
  1_2H_WT : Gain  Gain=1/(2*H_WT)  SaturateOnIntegerOverflow=on  OutDataTypeStr=Inherit: Same as input  ParamDataTypeStr=Inherit: Same as input
  Discrete-Time Integrator : DiscreteIntegrator  InitialCondition=w_wt0  SampleTime=Ts  ICPrevOutput=DiscIntNeverNeededParam  ICPrevScaledInput=DiscIntNeverNeededParam
  Discrete-Time Integrator1 : DiscreteIntegrator  InitialCondition=torque0/Ksh  SampleTime=Ts  ICPrevOutput=DiscIntNeverNeededParam  ICPrevScaledInput=DiscIntNeverNeededParam
  Mutual damping : Gain  Gain=D_mutual  SaturateOnIntegerOverflow=on  OutDataTypeStr=Inherit: Same as input  ParamDataTypeStr=Inherit: Same as input
  Stiffness : Gain  Gain=Ksh  SaturateOnIntegerOverflow=on  OutDataTypeStr=Inherit: Same as input  ParamDataTypeStr=Inherit: Same as input
  Sum : Sum  Inputs=+-  InputSameDT=on  SaturateOnIntegerOverflow=on  OutDataTypeStr=Inherit: Same as first input
  Sum1 : Sum  Inputs=+-  InputSameDT=on  SaturateOnIntegerOverflow=on  OutDataTypeStr=Inherit: Same as first input
  Sum2 : Sum  InputSameDT=on  SaturateOnIntegerOverflow=on  OutDataTypeStr=Inherit: Same as first input
  wbase : Gain  Gain=wbase  SaturateOnIntegerOverflow=on  OutDataTypeStr=Inherit: Same as input  ParamDataTypeStr=Inherit: Same as input
  W_wt (pu) : Outport  VectorParamsAs1DForOutWhenUnconnected=off
  T_shaft (pu) : Outport  Port=2  VectorParamsAs1DForOutWhenUnconnected=off
  wires:
  wbase/1 -> Discrete-Time Integrator1/1
  Discrete-Time Integrator1/1 -> Stiffness/1
  Stiffness/1 -> Sum2/1
  Sum/1 -> 1_2H_WT/1
  1_2H_WT/1 -> Discrete-Time Integrator/1
  Discrete-Time Integrator/1 -> Sum1/1, W_wt (pu)/1
  Generator speed (pu)/1 -> Sum1/2
  Sum1/1 -> wbase/1, Mutual damping/1
  Mutual damping/1 -> Sum2/2
  Sum2/1 -> Sum/2, T_shaft (pu)/1
  T_wt (pu)/1 -> Sum/1

== system WindFarmDFIG/DFIG Wind Turbine/Wind Turbine ==
  W_wt (pu) : Inport
  Pitch angle (deg) : Inport  Port=2
  Wind speed (m/s) : Inport  Port=3
  ->pu : Gain  Gain=1/Prated
  Avoid div. by zero : Saturate  UpperLimit=inf  LowerLimit=eps
  "Avoid div. by zero " : Saturate  UpperLimit=inf  LowerLimit=eps
  Fcn1 : Fcn  Expr=K1*u[2]/u[1]
  Fcn2 : Fcn  Expr=c1*(c6*u[1] + (-c4 - c3*(2.5 + u[2]) + c2*(1/(u[1] + c7*(2.5 + u[2])) -c8/(1 + (2.5 + u[2])^3)))/exp(c5*(1/(u[1] + c7*(2.5 + u[2])) - c8/(1 + (2.5 + u[2])^3))))
  "K2*Cp*wind^3 " : Fcn  Expr=K2*u[1]^3*u[2]
  Mux : Mux  Inputs=2
  Mux1 : Mux  Inputs=2
  Mux2 : Mux  Inputs=2
  Product2 : Product  Inputs=*/  InputSameDT=on  SaturateOnIntegerOverflow=on  OutDataTypeStr=Inherit: Same as first input
  Tt (pu) : Outport  VectorParamsAs1DForOutWhenUnconnected=off
  wires:
  "K2*Cp*wind^3 "/1 -> ->pu/1
  "Avoid div. by zero "/1 -> Product2/2, Mux/2
  Avoid div. by zero/1 -> Mux/1, Mux2/1
  W_wt (pu)/1 -> "Avoid div. by zero "/1
  Pitch angle (deg)/1 -> Mux1/2
  Mux2/1 -> "K2*Cp*wind^3 "/1
  Fcn2/1 -> Mux2/2  "Cp"
  Mux/1 -> Fcn1/1
  Mux1/1 -> Fcn2/1
  Fcn1/1 -> Mux1/1  "lambda"
  Wind speed (m/s)/1 -> Avoid div. by zero/1
  Product2/1 -> Tt (pu)/1
  ->pu/1 -> Product2/1  "power_pu"

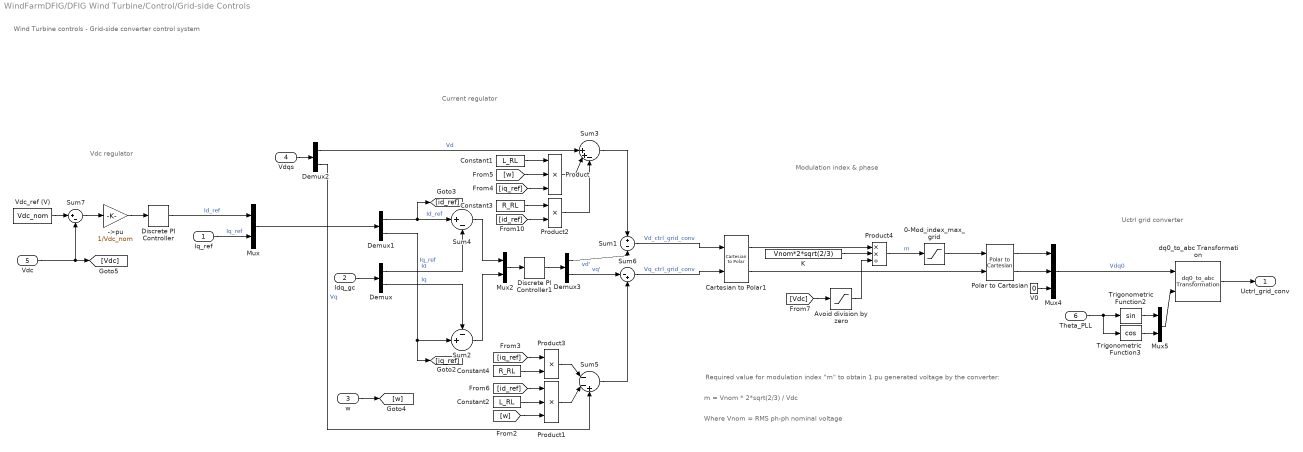
== system WindFarmDFIG/DFIG Wind Turbine/Control/Grid-side Controls ==
  note: Uctrl grid converter
  note: Modulation index & phase
  note: Current regulator
  note: Vdc regulator
  note: Required value for modulation index "m" to obtain 1 pu generated voltage by the converter:
  note: m = Vnom * 2*sqrt(2/3) / Vdc
  note: Where Vnom = RMS ph-ph nominal voltage
  note: Wind Turbine controls - Grid-side converter control system
  Iq_ref : Inport
  Idq_gc : Inport  Port=2
  w : Inport  Port=3
  Vdqs : Inport  Port=4
  Vdc : Inport  Port=5
  Theta_PLL : Inport  Port=6
  ->pu : Gain  Gain=1/Vdc_nom
  0-Mod_index_max_grid : Saturate  UpperLimit=Mod_index_max_grid  LowerLimit=0
  Avoid division by zero : Saturate  UpperLimit=inf  LowerLimit=1e-6
  Cartesian to Polar1 : simulink_extras/Transformations/Cartesian to Polar
  Constant1 : Constant  Value=L_RL
  Constant2 : Constant  Value=L_RL
  Constant3 : Constant  Value=R_RL
  Constant4 : Constant  Value=R_RL
  Demux{,1..3} (4 alike) : Demux  Outputs=2
      settings: DisplayOption=none
  Discrete PI Controller : powerlib_extras/Discrete  Control Blocks/Discrete PI Controller  Kp=Kp_dc  Ki=Ki_dc  Par_Limits=[1 -1]*Imax_grid_conv  Init=0  Ts=Ts
  Discrete PI Controller1 : powerlib_extras/Discrete  Control Blocks/Discrete PI Controller  Kp=Kp_grid_side_cur_reg  Ki=Ki_grid_side_cur_reg  Par_Limits=[1.0 -1.0] *Lim_grid_side_cur_reg  Init=0  Ts=Ts
  K : Constant  Value=Vnom*2*sqrt(2/3)
  Mux : Mux  Inputs=2
  Mux2 : Mux  Inputs=2
  Mux4 : Mux  Inputs=3
  Mux5 : Mux  Inputs=2
  Polar to Cartesian : simulink_extras/Transformations/Polar to Cartesian
  Product : Product  Inputs=3  InputSameDT=on  SaturateOnIntegerOverflow=on  OutDataTypeStr=Inherit: Same as first input
  Product1 : Product  Inputs=3  InputSameDT=on  SaturateOnIntegerOverflow=on  OutDataTypeStr=Inherit: Same as first input
  Product2 : Product  InputSameDT=on  SaturateOnIntegerOverflow=on  OutDataTypeStr=Inherit: Same as first input
  Product3 : Product  InputSameDT=on  SaturateOnIntegerOverflow=on  OutDataTypeStr=Inherit: Same as first input
  Product4 : Product  Inputs=**/  InputSameDT=on  SaturateOnIntegerOverflow=on  OutDataTypeStr=Inherit: Same as first input
  Sum1 : Sum  Inputs=+-  InputSameDT=on  SaturateOnIntegerOverflow=on  OutDataTypeStr=Inherit: Same as first input
  Sum2 : Sum  Inputs=-+|  InputSameDT=on  SaturateOnIntegerOverflow=on  OutDataTypeStr=Inherit: Same as first input
  Sum3 : Sum  Inputs=||++-  InputSameDT=on  SaturateOnIntegerOverflow=on  OutDataTypeStr=Inherit: Same as first input
  Sum4 : Sum  Inputs=|+-  InputSameDT=on  SaturateOnIntegerOverflow=on  OutDataTypeStr=Inherit: Same as first input
  Sum5 : Sum  Inputs=|--+  InputSameDT=on  SaturateOnIntegerOverflow=on  OutDataTypeStr=Inherit: Same as first input
  Sum6 : Sum  Inputs=|-+  InputSameDT=on  SaturateOnIntegerOverflow=on  OutDataTypeStr=Inherit: Same as first input
  Sum7 : Sum  Inputs=|+-  InputSameDT=on  SaturateOnIntegerOverflow=on  OutDataTypeStr=Inherit: Same as first input
  Trigonometric Function2 : Trigonometry
  Trigonometric Function3 : Trigonometry  Operator=cos
  V0 : Constant  Value=0
  Vdc_ref (V) : Constant  Value=Vdc_nom
  dq0_to_abc Transformation : powerlib_extras/Measurements/dq0_to_abc Transformation
  Uctrl_grid_conv : Outport  VectorParamsAs1DForOutWhenUnconnected=off
  wires:
  Sum6/1 -> Cartesian to Polar1/2  "Vq_ctrl_grid_conv"
  Sum1/1 -> Cartesian to Polar1/1  "Vd_ctrl_grid_conv"
  dq0_to_abc Transformation/1 -> Uctrl_grid_conv/1
  Theta_PLL/1 -> Trigonometric Function2/1, Trigonometric Function3/1
  Mux4/1 -> dq0_to_abc Transformation/1  "Vdq0"
  Polar to Cartesian/2 -> Mux4/2
  Polar to Cartesian/1 -> Mux4/1
  V0/1 -> Mux4/3
  Trigonometric Function3/1 -> Mux5/2
  Trigonometric Function2/1 -> Mux5/1
  Mux5/1 -> dq0_to_abc Transformation/2
  [Vdc] -> Avoid division by zero/1
  Product4/1 -> 0-Mod_index_max_grid/1  "m"
  K/1 -> Product4/2
  Avoid division by zero/1 -> Product4/3
  Cartesian to Polar1/1 -> Product4/1
  0-Mod_index_max_grid/1 -> Polar to Cartesian/1
  Cartesian to Polar1/2 -> Polar to Cartesian/2
  Mux/1 -> Demux1/1
  Idq_gc/1 -> Demux/1
  w/1 -> [w]
  Constant2/1 -> Product1/2
  Discrete PI Controller1/1 -> Demux3/1
  Mux2/1 -> Discrete PI Controller1/1
  Demux2/1 -> Sum3/1  "Vd"
  Constant1/1 -> Product/1
  Vdqs/1 -> Demux2/1
  Demux/2 -> Sum2/1  "Iq"
  Demux/1 -> Sum4/2  "Id"
  Product/1 -> Sum3/2
  Constant3/1 -> Product2/1
  Constant4/1 -> Product3/2
  Product1/1 -> Sum5/2
  Demux2/2 -> Sum5/3  "Vq"
  Product2/1 -> Sum3/3
  Product3/1 -> Sum5/1
  Sum4/1 -> Mux2/1
  Sum2/1 -> Mux2/2
  [w] -> Product1/3
  [w] -> Product/2
  [iq_ref] -> Product/3
  [id_ref] -> Product2/2
  [iq_ref] -> Product3/1
  [id_ref] -> Product1/1
  Demux3/1 -> Sum1/2  "vd'"
  Demux3/2 -> Sum6/1  "vq'"
  Demux1/2 -> [iq_ref], Sum2/2  "Iq_ref"
  Demux1/1 -> Sum4/1, [id_ref]  "Id_ref"
  Sum3/1 -> Sum1/1
  Sum5/1 -> Sum6/2
  Discrete PI Controller/1 -> Mux/1  "Id_ref"
  Sum7/1 -> ->pu/1
  ->pu/1 -> Discrete PI Controller/1
  Vdc/1 -> [Vdc], Sum7/2
  Iq_ref/1 -> Mux/2  "Iq_ref"
  Vdc_ref (V)/1 -> Sum7/1
